simulink model "thermal_control"  (R2026a)
settings: Solver=ode45  StopTime=1800  MaxStep=1  RelTol=1e-4
values from neighbouring files (symbols this model uses):
  C_th = tau * P / K    (= 400)    [init_params.m]
  L = 3    [init_params.m]    (also in tune_pi.m)
  P = 50    [init_params.m]
  T_amb = 25    [init_params.m]
libraries: slpidlib x1
settings Model: Creator=Fufal Jigar  LastModifiedBy=Fufal Jigar

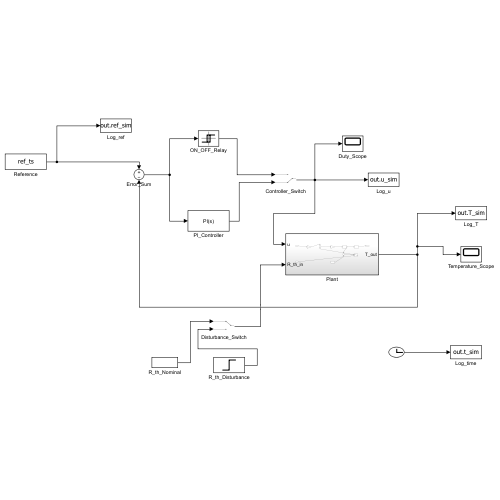
[thumbnail: Simulink's stored preview of the top-level diagram]
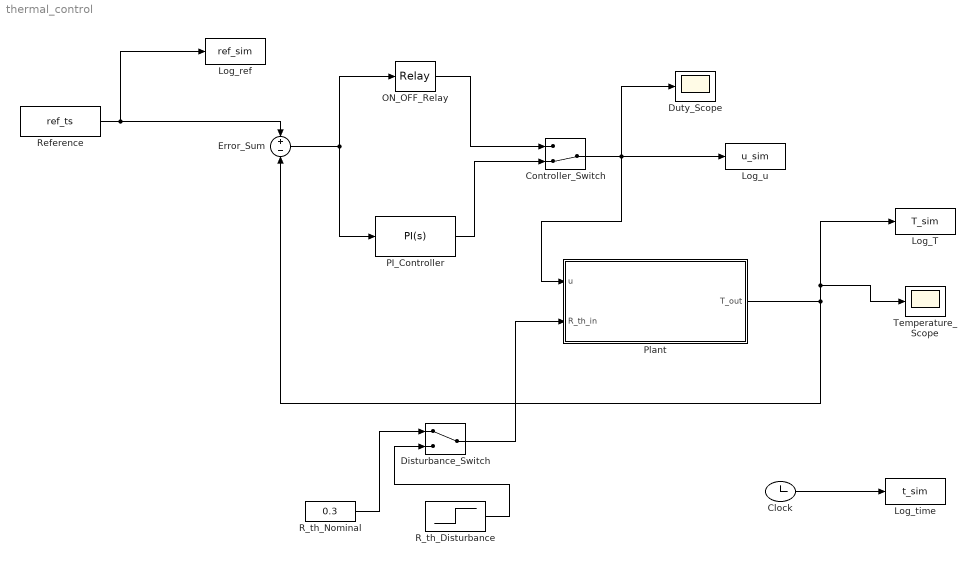
== system thermal_control ==
  Clock : Clock
  Controller_Switch : ManualSwitch  CurrentSetting=0
  Disturbance_Switch : ManualSwitch
  Duty_Scope : Scope
      settings: ActiveDisplayYMinimum=-3.9876718914011349  ActiveDisplayYMaximum=18.659064193327517
  Error_Sum : Sum  Inputs=+-
  Log_T : ToWorkspace  VariableName=T_sim  SaveFormat=Timeseries  SampleTime=-1
  Log_ref : ToWorkspace  VariableName=ref_sim  SaveFormat=Timeseries  SampleTime=-1
  Log_time : ToWorkspace  VariableName=t_sim  SaveFormat=Timeseries  SampleTime=-1
  Log_u : ToWorkspace  VariableName=u_sim  SaveFormat=Timeseries  SampleTime=-1
  ON_OFF_Relay : Relay  OnSwitchValue=0.5  OffSwitchValue=-0.5
  PI_Controller : slpidlib/PID Controller  Controller=PI  Form=Parallel  TimeDomain=Continuous-time  UseExternalTs=off  SampleTime=-1  IntegratorMethod=Forward Euler  FilterMethod=Forward Euler  ControllerParametersSource=internal  P=0.53333  I=0.0044444  UseKiTs=off  D=0  UseExternalDerivativeSource=off  N=100  UseFilter=on  TunerSelectOption=Transfer Function Based (PID Tuner App)  InitialConditionSource=internal  InitialConditionForIntegrator=0  InitialConditionForFilter=0  DifferentiatorICPrevScaledInput=0  ExternalReset=none  TrackingMode=off  Kt=1  LimitOutput=off  SatLimitsSource=internal  UpperSaturationLimit=1  LowerSaturationLimit=0  LinearizeAsGain=on  AntiWindupMode=clamping  Kb=1  LimitIntegrator=off  UpperIntegratorSaturationLimit=inf  LowerIntegratorSaturationLimit=-inf  POutMin=[]  POutMax=[]  IOutMin=[]  IOutMax=[]  DOutMin=[]  DOutMax=[]  NOutMin=[]  NOutMax=[]  SumOutMin=[]  SumOutMax=[]  SaturationOutMin=[]  SaturationOutMax=[]  PParamMin=[]  PParamMax=[]  IParamMin=[]  IParamMax=[]  DParamMin=[]  DParamMax=[]  NParamMin=[]  NParamMax=[]  KbParamMin=[]  KbParamMax=[]  KtParamMin=[]  KtParamMax=[]  KbOutMin=[]  KbOutMax=[]  KtOutMin=[]  KtOutMax=[]  IntegratorOutMin=[]  IntegratorOutMax=[]  FilterOutMin=[]  FilterOutMax=[]  SumI1OutMin=[]  SumI1OutMax=[]  SumI2OutMin=[]  SumI2OutMax=[]  SumI3OutMin=[]  SumI3OutMax=[]  SumI4OutMin=[]  SumI4OutMax=[]  SumDOutMin=[]  SumDOutMax=[]  DifferentiatorOutMin=[]  DifferentiatorOutMax=[]  FilterDiffOutCoefMin=[]  FilterDiffOutCoefMax=[]  ReciprocalOutMin=[]  ReciprocalOutMax=[]  SumDenOutMin=[]  SumDenOutMax=[]  SumNumOutMin=[]  SumNumOutMax=[]  DivideOutMin=[]  DivideOutMax=[]  UdiffTsProdOutMin=[]  UdiffTsProdOutMax=[]  NTsProdOutMin=[]  NTsProdOutMax=[]  UintegralTsProdOutMin=[]  UintegralTsProdOutMax=[]  UngainTsProdOutMin=[]  UngainTsProdOutMax=[]  ClampingZeroOutDataTypeStr=Inherit: Inherit via back propagation  ClampingZeroOutMin=[]  ClampingZeroOutMax=[]  FilterDenConstantOutDataTypeStr=Inherit: Inherit via back propagation  FilterDenConstantOutMin=[]  FilterDenConstantOutMax=[]  PCopyOutDataTypeStr=Inherit: Inherit via back propagation  PCopyOutMin=[]  PCopyOutMax=[]  NCopyOutDataTypeStr=Inherit: Inherit via back propagation  NCopyOutMin=[]  NCopyOutMax=[]  IntegratorContinuousStateAttributes=''  IntegratorStateMustResolveToSignalObject=off  IntegratorRTWStateStorageClass=Auto  FilterContinuousStateAttributes=''  FilterStateMustResolveToSignalObject=off  FilterRTWStateStorageClass=Auto  ParallelPVariant=InternalParameters  IdealPVariant=Disabled  IVariant=InternalParameters  DVariant=Disabled  IntegratorVariant=Continuous  SatVariant=Disabled  AWVariant=Passthrough  PCopyVariant=Disabled  TRVariant=Disabled  FdbkBlocksVariant=Forward  IdealPFdbkVariant=Disabled  SatFdbkVariant=Disabled  DerivativeFilterVariant=Disabled  NVariant=Disabled  NCopyVariant=Disabled_SignalSpec  FilterICVariant=Disabled  IntegratorICVariant=InternalICs  ExternalResetVariant=Disabled  TRSumVariant=Passthrough  SumFdbkVariant=Disabled  SumVariant=Sum_PI  TsampFilterVariant=InternalTs  TsampNgainVariant=Passthrough  TsampIntegralVariant=Disabled_SignalSpec  ExternalSaturationOutDataTypeStr=Inherit: Same as second input  DerivativeSourceVariant=Disabled  PreIntVariant=InternalPreInt
  Plant : Subsystem
  R_th_Disturbance : Step  Time=900  InitialValue=0.3  FinalValue=0.39  SampleTime=0
  R_th_Nominal : Constant  Value=0.3
  Reference : FromWorkspace  VariableName=ref_ts  OutputAfterFinalValue=Holding final value
  Temperature_Scope : Scope
      settings: ActiveDisplayYMinimum=-4.9999999950560534  ActiveDisplayYMaximum=44.999999955504492
  wires:
  Reference/1 -> Error_Sum/1, Log_ref/1
  Error_Sum/1 -> PI_Controller/1, ON_OFF_Relay/1
  ON_OFF_Relay/1 -> Controller_Switch/1
  PI_Controller/1 -> Controller_Switch/2
  Controller_Switch/1 -> Duty_Scope/1, Plant/1(u), Log_u/1
  R_th_Nominal/1 -> Disturbance_Switch/1
  R_th_Disturbance/1 -> Disturbance_Switch/2
  Disturbance_Switch/1 -> Plant/2(R_th_in)
  Plant/1(T_out) -> Error_Sum/2, Log_T/1, Temperature_Scope/1
  Clock/1 -> Log_time/1

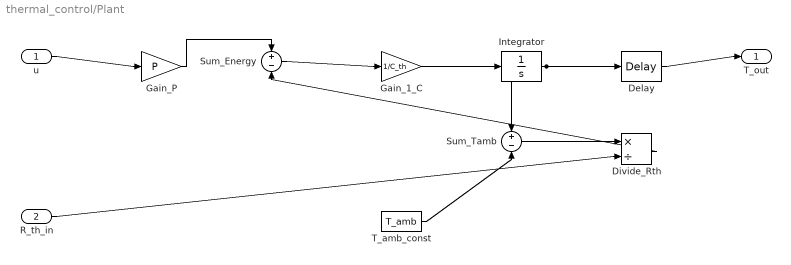
== system thermal_control/Plant ==
  u : Inport
  R_th_in : Inport  Port=2
  Delay : TransportDelay  DelayTime=L
  Divide_Rth : Product  Inputs=*/
  Gain_1_C : Gain  Gain=1/C_th
  Gain_P : Gain  Gain=P
  Integrator : Integrator  InitialCondition=T_amb
  Sum_Energy : Sum  Inputs=+-
  Sum_Tamb : Sum  Inputs=+-
  T_amb_const : Constant  Value=T_amb
  T_out : Outport
  wires:
  u/1 -> Gain_P/1
  Gain_P/1 -> Sum_Energy/1
  Sum_Energy/1 -> Gain_1_C/1
  Gain_1_C/1 -> Integrator/1
  Integrator/1 -> Delay/1, Sum_Tamb/1
  Delay/1 -> T_out/1
  T_amb_const/1 -> Sum_Tamb/2
  Sum_Tamb/1 -> Divide_Rth/1
  R_th_in/1 -> Divide_Rth/2
  Divide_Rth/1 -> Sum_Energy/2
